simulink model "PMSM_FOC_R2026a"  (R2026a)
settings: Solver=ode4  StopTime=0.25  FixedStep=timing_h  MaxStep=1e-6
InitFcn:
  | pmsm_sensorless_v2_init(bdroot);
model workspace (MATLAB code in the model file + MAT data in the model file):
  T = 1e-6    (= 1e-06)
  MotorProfile = 'CHENSHA 200W / firmware profile revision 2'
  MotorSourceCommit = '48d6e86814ac6657b1313b4c92ef24c88f492e07'
  Pn = 200
  Un = 24
  Vdc = 24
  I_rated_rms = 11.5
  I_peak_rms = 23
  In = sqrt(2)*I_rated_rms
  I_peak = sqrt(2)*I_peak_rms
  n = 3000
  p = 5
  Rs = 0.105125
  Ld = 103.7615e-6    (= 0.0001037615)
  Lq = 103.7615e-6    (= 0.0001037615)
  Ls = Ld    (= 0.0001037615)
  phis = 0.06/(sqrt(2)*1.5*p)
  J = 32e-6    (= 3.2e-05)
  F = 0
  Kt = 1.5*p*phis
  Tn = 0.69
  T_peak = 1.38
  Iq_limit = 8
  accel_limit_rad_s2 = 1200
  speed_peak_rad_s = 335
  I_protection_A = 10
  Vbus_protection_high_V = 30
  Vbus_protection_low_V = 10
  RE = 10000
  rr = 2*pi/RE    (= 0.000628318530718)
  encoder_direction = -1
  fN = p*n/60    (= 250)
  wN = 2*pi*fN    (= 1570.79632679)
  ki_p = 0.8
  ki_i = 1
  fc = 20e3    (= 20000)
  Ts = 1/fc    (= 5e-05)
  dt = Ts    (= 5e-05)
  Ts_speed = 2*dt    (= 0.0001)
  w_sb = 2*pi*fN*1.2    (= 1884.95559215)
  fcb = 1000
  fwb = 50
  wc = 2*pi*fcb    (= 6283.18530718)
  wsc = 2*pi*fwb    (= 314.159265359)
  K = 30/pi    (= 9.54929658551)
  kp_w = 0.00069087230807625508    (= 0.000690872308076)
  ki_w = 0.04340878735241975    (= 0.0434087873524)
  ks_w = 0.98718608264211138    (= 0.987186082642)
  kp_id = 0.7539822368615503    (= 0.753982236862)
  ki_id = 879.64594300514204    (= 879.645943005)
  ks_id = 1.1309733552923253    (= 1.13097335529)
  kp_iq = 0.7539822368615503    (= 0.753982236862)
  ki_iq = 879.64594300514204    (= 879.645943005)
  ks_iq = 1.1309733552923253    (= 1.13097335529)
  Bm = 0
  uplimit_w = Kt*Iq_limit
  downlimit_w = -uplimit_w
  uplimit_id = Vdc/sqrt(3)
  downlimit_id = -uplimit_id
  uplimit_iq = Vdc/sqrt(3)
  downlimit_iq = -uplimit_iq
  teaching_Ts_speed = Ts_speed    (= 0.0001)
  teach_pwm_on = 0
  teach_pwm_cycles = 1
  decoupling_enabled = 1
  voltage_utilization = 0.96
  timing_on = 0
  timing_h = 1e-6    (= 1e-06)
  timing_control_sample = dt    (= 5e-05)
  timing_speed_sample = Ts_speed    (= 0.0001)
  timing_static_math = -1
  timing_carrier_y = [0 Ts/2 0]
  timing_adc_cfg = [0 0 0 1e-6 Ts 24.375e-6 1.1875e-6 1.5e-6 0 .5e-6 2]
  timing_pwm_cfg = [0 1e-6 Ts 24.375e-6 1.1875e-6 1.5e-6 0 5e-6 0 4000]
  dead_gate_on = 0
  dead_h = 1e-6    (= 1e-06)
  dead_gate_cfg = [0 1e-6 .5e-6]
  dead_comp_cfg = [0 .5e-6 Ts .05]
  dead_bridge_cfg = [p phis .01 0 .01 .7]
  sless_adc_mode = [1 0]
  sless_cfg = [0.105125 0.0001037615 5e-05 0.950604638176 0.469872645179 70 14 0.2 0.028048810878 0.777767679172 533.065441461 142122.303376 ... (18 elements, 1x18)]
  sless_direction = 1
  sless_enabled = 1
  sless_v2_cfg = [6.25e-08 5e-05 0.0001 2.4375e-05 1.1875e-06 1.5e-06 0 0 3e-06 5e-06 2e-06 6e-05 ... (35 elements, 1x35)]
  sless_v2_interference_s = 0
  sless_voltage_cfg = [6.25e-08 5e-05 2.8875e-05 0.105125 0.0001037615 1]
undefined symbols (not defined in the file): DiscIntNeverNeededParam
libraries: simulink x3
(part 3 of 3)

== matlab function PMSM_FOC_R2026a/SVPWM Function v1.0 ==
  data: alpha input; beta input; Vdc input; Ts input; Tcm output; sector output; diagnostic output
function [Tcm,sector,diagnostic] = fcn(alpha,beta,Vdc,Ts)
% Original six-sector construction, with simultaneous overmodulation scaling.
% Tcm is a threshold in [0,Ts/2]; upper duty = 1-2*Tcm/Ts.
% diagnostic: t1,t2,total zero-vector time,Da,Db,Dc,overmodulated,bounds_guard.
Tcm=ones(1,3)*Ts/4;sector=0;
diagnostic=[0 0 Ts .5 .5 .5 0 0];
if Vdc<=0 || Ts<=0 || (alpha==0 && beta==0),return;end
ref1=beta;ref2=(-beta+sqrt(3)*alpha)/2;ref3=(-beta-sqrt(3)*alpha)/2;
sector=4*double(ref3>0)+2*double(ref2>0)+double(ref1>0);
X=Ts*sqrt(3)/Vdc*beta;
Y=Ts*sqrt(3)/Vdc*(sqrt(3)*alpha+beta)/2;
Z=Ts*sqrt(3)/Vdc*(-sqrt(3)*alpha+beta)/2;
switch sector
 case 1,t1=Z;t2=Y;
 case 2,t1=Y;t2=-X;
 case 3,t1=-Z;t2=X;
 case 4,t1=-X;t2=Z;
 case 5,t1=X;t2=-Y;
 otherwise,t1=-Y;t2=-Z;
end
t1=max(0,t1);t2=max(0,t2);
total=t1+t2;over=double(total>Ts);
if total>Ts
 scale=Ts/total;t1=t1*scale;t2=t2*scale;
end
tzero=max(0,Ts-t1-t2);
ta=tzero/4;tb=ta+t1/2;tc=tb+t2/2;
switch sector
 case 1,Tcm=[tb ta tc];
 case 2,Tcm=[ta tc tb];
 case 3,Tcm=[ta tb tc];
 case 4,Tcm=[tc tb ta];
 case 5,Tcm=[tc ta tb];
 case 6,Tcm=[tb tc ta];
end
guard=double(any(Tcm<-1e-12) || any(Tcm>Ts/2+1e-12));
Tcm=min(Ts/2,max(0,Tcm));
diagnostic=[t1 t2 tzero 1-2*Tcm/Ts over guard];
end

== matlab function PMSM_FOC_R2026a/输出延迟/CCR预装载 ==
  settings: updateMethod=DISCRETE  sampleTime=timing_h
  data: t input; applied output size=[1 3]; request input; cfg input; diag output size=[1 12]
function [applied,diag] = timing_pwm(t,request,cfg)
%#codegen
% cfg: on, h, Ts, trigger, aperture, rank, sync, compute, update mode, ARR.
% mode=0: RCR=0 update at both extrema; mode=1: underflow-only comparison.
% If a write coincides with UEV, UEV wins and the new CCR waits for the next UEV.
persistent shadow active pending shadow_seq active_seq writes stamp delay
if isempty(shadow)
 shadow=cfg(3)/4*ones(1,3);active=shadow;pending=false;
 shadow_seq=0;active_seq=0;writes=0;stamp=0;delay=0;
end
applied=active;diag=zeros(1,12);
if cfg(1)==0,return;end
h=cfg(2);N=round(cfg(3)/h);tick=round(t/h);phase=mod(tick,N);
jeos=round((cfg(4)+cfg(7)+3*cfg(6))/h);wr=jeos+round(cfg(8)/h);
update=(phase==0 || (cfg(9)==0 && phase==N/2));write=(phase==wr);
latched=false;
if update && pending
 active=shadow;active_seq=shadow_seq;pending=false;latched=true;delay=t-stamp;
end
if write
 duty=max(0,min(1,1-2*reshape(request,1,3)/cfg(3)));
 ccr=floor(duty*cfg(10)+1e-9);
 shadow=cfg(3)/2*(1-ccr/cfg(10));shadow_seq=shadow_seq+1;
 writes=writes+1;pending=true;stamp=floor(tick/N)*cfg(3)+jeos*h;
end
applied=active;
cnt=2*min(phase,N-phase)/N*cfg(10);
diag=[cnt double(phase>=N/2) double(update) double(write) double(latched) ...
 shadow_seq active_seq double(pending) delay shadow];
end

== matlab function PMSM_FOC_R2026a/Universal Bridge/门极死区 ==
  settings: updateMethod=DISCRETE  sampleTime=dead_h
  data: t input; gates output size=[1 6]; request input; cfg input; blank output size=[1 3]
function [gates,blank] = gate_deadtime(t,request,cfg)
%#codegen
% cfg = [enable, event grid, programmed deadtime]. Fall immediately;
% delay each rising edge. A pulse shorter than deadtime is suppressed.
persistent previous rise armed active
if isempty(previous)
 previous=zeros(1,6);rise=zeros(1,6);armed=false(1,6);active=zeros(1,6);
end
r=double(reshape(request,1,6)>0.5);gates=r;blank=zeros(1,3);
if cfg(1)==0,return;end
assert(all(r(1:2:5)+r(2:2:6)<=1));
tick=round(t/cfg(2));delay=round(cfg(3)/cfg(2));
for k=1:6
 if r(k)==0
  active(k)=0;armed(k)=false;
 elseif previous(k)==0
  rise(k)=tick;armed(k)=true;active(k)=0;
 end
 if armed(k)&&tick-rise(k)>=delay,active(k)=1;armed(k)=false;end
end
previous=r;gates=active;
assert(all(gates(1:2:5)+gates(2:2:6)<=1));
blank=1-gates(1:2:5)-gates(2:2:6);
end

== matlab function PMSM_FOC_R2026a/Universal Bridge/续流 ==
  settings: updateMethod=CONTINUOUS
  data: gates input; phase output size=[1 3]; state input; Vdc input; cfg input; diagnostic output size=[1 9]
function [phase,diagnostic] = bridge_freewheel(gates,state,Vdc,cfg)
%#codegen
% Static switched bridge for the present non-salient floating-star PMSM.
% cfg = [pole pairs, flux, zero-current band, drop enable, Ron, Vf].
% Positive current flows from pole to motor. During both-OFF, positive
% current uses the lower diode; negative current uses the upper diode.
x=reshape(state,1,4);g=reshape(gates,1,6);bus=max(Vdc,0);
theta=cfg(1)*x(4)+[0 -2*pi/3 2*pi/3];
current=x(1)*cos(theta)-x(2)*sin(theta);
emf=-cfg(1)*x(3)*cfg(2)*sin(theta);
pole=zeros(1,3);path=zeros(1,3);fixed=false(1,3);
ron=cfg(4)*cfg(5);vf=cfg(4)*cfg(6);
for k=1:3
 hi=g(2*k-1)>0.5;lo=g(2*k)>0.5;assert(~(hi&&lo));
 if hi,pole(k)=bus/2-ron*current(k);fixed(k)=true;
 elseif lo,pole(k)=-bus/2-ron*current(k);fixed(k)=true;
 elseif current(k)>cfg(3),pole(k)=-bus/2-vf;path(k)=-1;fixed(k)=true;
 elseif current(k)<-cfg(3),pole(k)=bus/2+vf;path(k)=1;fixed(k)=true;
 end
end
% Near zero, a disconnected phase follows its open-circuit EMF until a
% diode rail is reached. Small current band is a declared numerical model,
% not a device capacitance or exact diode complementarity solver.
neutral=0;
for pass=1:4
 count=sum(double(fixed));if count>0,neutral=sum((pole-emf).*double(fixed))/count;end
 changed=false;
 for k=1:3
  if ~fixed(k)
   pole(k)=emf(k)+neutral;
   if pole(k)>bus/2+vf,pole(k)=bus/2+vf;path(k)=1;fixed(k)=true;changed=true;
   elseif pole(k)<-bus/2-vf,pole(k)=-bus/2-vf;path(k)=-1;fixed(k)=true;changed=true;
   end
  end
 end
 if ~changed,break;end
end
% For near-zero open phases the neutral above enforces zero derivative;
% all fixed phases satisfy the usual floating-star mean subtraction.
phase=pole-sum(pole)/3;
diagnostic=[path pole current];
end

== matlab function PMSM_FOC_R2026a/限压/死区补偿 ==
  settings: updateMethod=DISCRETE  sampleTime=timing_control_sample
  data: current input; dq output size=[1 2]; theta input; Vdc input; cfg input; diagnostic output size=[1 8]
function [dq,diagnostic] = deadtime_comp(current,theta,Vdc,cfg)
%#codegen
% cfg = [enable, compensated deadtime, PWM period, current hysteresis].
% Uses measured current ONLY. Positive phase current needs positive voltage
% correction. Correction enters BEFORE the existing final dq circle limit.
persistent polarity
if isempty(polarity),polarity=zeros(1,3);end
dq=zeros(1,2);diagnostic=zeros(1,8);
if cfg(1)==0,return;end
i=reshape(current,1,3);
for k=1:3
 if i(k)>cfg(4),polarity(k)=1;
 elseif i(k)<-cfg(4),polarity(k)=-1;
 end
end
abc=max(Vdc,0)*cfg(2)/cfg(3)*polarity;abc=abc-sum(abc)/3;
alpha=(2*abc(1)-abc(2)-abc(3))/3;beta=(abc(2)-abc(3))/sqrt(3);
dq=[alpha*cos(theta)+beta*sin(theta),-alpha*sin(theta)+beta*cos(theta)];
diagnostic=[abc dq polarity];
end

== matlab function PMSM_FOC_R2026a/无感观测/采样输入/校准对齐 ==
  settings: updateMethod=DISCRETE  sampleTime=timing_control_sample
  data: t input double size=1; current output double size=[2 1]; measured input double size=[3 1]; adc input double size=[3 1]; diag input double size=[1 15]; cfg input double size=[1 35]; calibrated output double size=[3 1]; valid output boolean size=1; adc_valid output boolean size=1; timing_valid output boolean size=1; meta output double size=[12 1]
function [current,calibrated,valid,adc_valid,timing_valid,meta]=sless_v2_measure_block(t,measured,adc,diag,cfg)
%#codegen
persistent s
if isempty(s),s=sensorless_v2_measure_state;end
c=sensorless_v2_config_rt(cfg);
[s,current,calibrated,valid,adc_valid,timing_valid,meta]=sensorless_v2_measure_step(s,t,measured,adc,diag,c);
end
